simulink model "rocket_rcs"  (R2024a)
settings: Solver=FixedStepAuto  StartTime=0.0001  StopTime=140  FixedStep=0.0001  RelTol=1e-3
undefined symbols (not defined in the file or in its folder): deg, Earth, rad, s, WGS84
libraries: aerolibconvert2 x26, matrix_library x5, eePwmGenerator x5, slpidlib x5, aerolibasang x2, simulink x2, sharedtransform x1, aerolibtransform2 x1, shared6dof x1
(part 2 of 2)

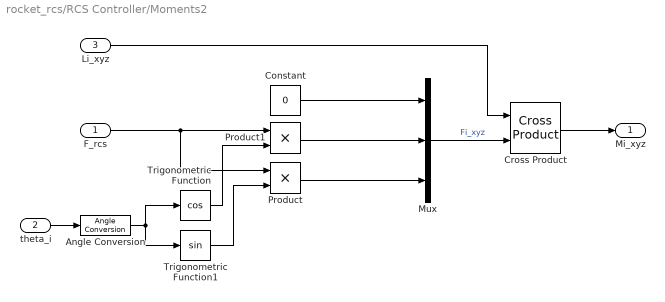
== system rocket_rcs/RCS Controller/Moments2 ==
  F_rcs : Inport
  theta_i : Inport  Port=2
  Li_xyz : Inport  Port=3
  Angle Conversion : aerolibconvert2/Angle Conversion  IU=deg  OU=rad
  Constant : Constant  Value=0
  Cross Product : matrix_library/Cross Product
  Mux : Mux  Inputs=3
  Product : Product
  Product1 : Product
  Trigonometric Function : Trigonometry  Operator=cos
  Trigonometric Function1 : Trigonometry
  Mi_xyz : Outport
  wires:
  Product1/1 -> Mux/2
  Product/1 -> Mux/3
  F_rcs/1 -> Product/1, Product1/1
  Trigonometric Function/1 -> Product1/2
  Trigonometric Function1/1 -> Product/2
  Constant/1 -> Mux/1
  Mux/1 -> Cross Product/2  "Fi_xyz"
  Li_xyz/1 -> Cross Product/1
  Cross Product/1 -> Mi_xyz/1
  theta_i/1 -> Angle Conversion/1
  Angle Conversion/1 -> Trigonometric Function1/1, Trigonometric Function/1

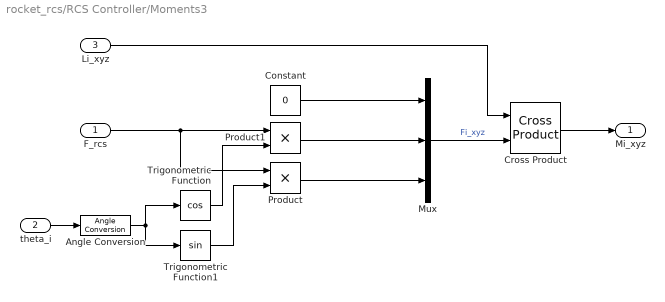
== system rocket_rcs/RCS Controller/Moments3 ==
  F_rcs : Inport
  theta_i : Inport  Port=2
  Li_xyz : Inport  Port=3
  Angle Conversion : aerolibconvert2/Angle Conversion  IU=deg  OU=rad
  Constant : Constant  Value=0
  Cross Product : matrix_library/Cross Product
  Mux : Mux  Inputs=3
  Product : Product
  Product1 : Product
  Trigonometric Function : Trigonometry  Operator=cos
  Trigonometric Function1 : Trigonometry
  Mi_xyz : Outport
  wires:
  Product1/1 -> Mux/2
  Product/1 -> Mux/3
  F_rcs/1 -> Product/1, Product1/1
  Trigonometric Function/1 -> Product1/2
  Trigonometric Function1/1 -> Product/2
  Constant/1 -> Mux/1
  Mux/1 -> Cross Product/2  "Fi_xyz"
  Li_xyz/1 -> Cross Product/1
  Cross Product/1 -> Mi_xyz/1
  theta_i/1 -> Angle Conversion/1
  Angle Conversion/1 -> Trigonometric Function1/1, Trigonometric Function/1

== system rocket_rcs/RCS Controller/PWM示例 ==
  Abs1 : Abs  SaturateOnIntegerOverflow=off
  Dead Zone2 : DeadZone  LowerValue=-0.05  UpperValue=0.05
  Divide : Product  Inputs=*/
  Dot Product : DotProduct  OutDataTypeStr=Inherit: Inherit via internal rule
  Dot Product1 : DotProduct  OutDataTypeStr=Inherit: Inherit via internal rule
  Mrcs : Constant  Value=490
  PWM Generator : eePwmGenerator/PWM Generator  CarrCount=Up  Tper=0.2  Tdelay=0  Ts=0
  Saturation : Saturate  UpperLimit=1  LowerLimit=-1
  Sign : Signum
  Sine Wave1 : Sin  Amplitude=490  Frequency=pi/2  SampleTime=0
  wires:
  Sine Wave1/1 -> Sign/1, Divide/1  "Mc"
  Sign/1 -> Dot Product/1
  Dot Product/1 -> Dot Product1/2
  Saturation/1 -> PWM Generator/1
  PWM Generator/1 -> Dot Product1/1  "PWM"
  Abs1/1 -> Dead Zone2/1
  Mrcs/1 -> Dot Product/2, Divide/2
  Divide/1 -> Abs1/1
  Dead Zone2/1 -> Saturation/1

== matlab function rocket_rcs/RCS Controller/RCS select1 ==
  data: dm_roll input; u1 output; u2 output; u3 output; u4 output; dm_pitch input; dm_raw input
% RCS 喷管选择逻辑：查表控制
function [u1,u2,u3,u4] = RCSselect(dm_roll, dm_pitch, dm_raw)

if dm_pitch < 0 && dm_raw < 0 && dm_roll < 0
    u1 = 0;
    u2 = 1;
    u3 = 1;
    u4 = 1;
elseif dm_pitch < 0 && dm_raw < 0 && dm_roll == 0
    u1 = 0;
    u2 = 0;
    u3 = 0;
    u4 = 1;
elseif dm_pitch < 0 && dm_raw < 0 && dm_roll > 0
    u1 = 0;
    u2 = 0;
    u3 = 0;
    u4 = 1;
elseif dm_pitch < 0 && dm_raw == 0 && dm_roll < 0
    u1 = 0;
    u2 = 1;
    u3 = 0;
    u4 = 0;
elseif dm_pitch < 0 && dm_raw == 0 && dm_roll == 0
    u1 = 0;
    u2 = 1;
    u3 = 0;
    u4 = 1;
elseif dm_pitch < 0 && dm_raw == 0 && dm_roll > 0
    u1 = 0;
    u2 = 0;
    u3 = 0;
    u4 = 1;
elseif dm_pitch < 0 && dm_raw > 0 && dm_roll < 0
    u1 = 0;
    u2 = 1;
    u3 = 0;
    u4 = 0;
elseif dm_pitch < 0 && dm_raw > 0 && dm_roll == 0
    u1 = 0;
    u2 = 1;
    u3 = 0;
    u4 = 0;
elseif dm_pitch < 0 && dm_raw > 0 && dm_roll > 0
    u1 = 1;
    u2 = 1;
    u3 = 0;
    u4 = 1;

elseif dm_pitch == 0 && dm_raw < 0 && dm_roll < 0
    u1 = 0;
    u2 = 0;
    u3 = 1;
    u4 = 0;
elseif dm_pitch == 0 && dm_raw < 0 && dm_roll == 0
    u1 = 0;
    u2 = 0;
    u3 = 1;
    u4 = 1;
elseif dm_pitch == 0 && dm_raw < 0 && dm_roll > 0
    u1 = 0;
    u2 = 0;
    u3 = 0;
    u4 = 1;
elseif dm_pitch == 0 && dm_raw == 0 && dm_roll < 0
    u1 = 0;
    u2 = 1;
    u3 = 1;
    u4 = 0;    
elseif dm_pitch == 0 && dm_raw == 0 && dm_roll > 0
    u1 = 1;
    u2 = 0;
    u3 = 0;
    u4 = 1;  
elseif dm_pitch == 0 && dm_raw > 0 && dm_roll < 0
    u1 = 0;
    u2 = 1;
    u3 = 0;
    u4 = 0;
elseif dm_pitch == 0 && dm_raw > 0 && dm_roll == 0
    u1 = 1;
    u2 = 1;
    u3 = 0;
    u4 = 0;    
elseif dm_pitch == 0 && dm_raw > 0 && dm_roll > 0
    u1 = 1;
    u2 = 0;
    u3 = 0;
    u4 = 0;

elseif dm_pitch > 0 && dm_raw < 0 && dm_roll < 0
    u1 = 0;
    u2 = 0;
    u3 = 1;
    u4 = 0;
elseif dm_pitch > 0 && dm_raw < 0 && dm_roll == 0
    u1 = 0;
    u2 = 0;
    u3 = 1;
    u4 = 0;
elseif dm_pitch > 0 && dm_raw < 0 && dm_roll > 0
    u1 = 1;
    u2 = 0;
    u3 = 1;
    u4 = 1;
elseif dm_pitch > 0 && dm_raw == 0 && dm_roll < 0
    u1 = 0;
    u2 = 0;
    u3 = 1;
    u4 = 0;
elseif dm_pitch > 0 && dm_raw == 0 && dm_roll == 0
    u1 = 1;
    u2 = 0;
    u3 = 1;
    u4 = 0;
elseif dm_pitch > 0 && dm_raw == 0 && dm_roll > 0
    u1 = 1;
    u2 = 0;
    u3 = 0;
    u4 = 0;
elseif dm_pitch > 0 && dm_raw > 0 && dm_roll < 0
    u1 = 1;
    u2 = 1;
    u3 = 1;
    u4 = 0;
elseif dm_pitch > 0 && dm_raw > 0 && dm_roll == 0
    u1 = 1;
    u2 = 0;
    u3 = 0;
    u4 = 0;
elseif dm_pitch > 0 && dm_raw > 0 && dm_roll > 0
    u1 = 1;
    u2 = 0;
    u3 = 0;
    u4 = 0;

else
    u1 = 0;
    u2 = 0;
    u3 = 0;
    u4 = 0;

end
end

== matlab function rocket_rcs/AeroDynamics/Air Density ==
  data: h input; Rho output
function Rho = density(h)
% rho0 = 1.225;
T0 = 288.15;    % K
p0 = 101325;   % Pa
R = 287.04;
T11 = 216.65;
p11 = 22632;
h11 = 11000;
g = 9.81;

if h <= 11000
    T=T0 - 0.0065 * h;
    p = p0 * (1-0.0065*(h/T0))^5.2561;
    Rho = p / (R * T);

elseif h>11000 && h<=20000
    T = 216.65;
    p = p11 * exp(g*(h11 - h)/(R*T11));
    Rho = p / (R * T);

else
    T=216.65+0.001*(h-20000);
    Rho=0.088035*(T/216.65)^-35.1632;
end
end

== matlab function rocket_rcs/AeroDynamics/MATLAB Function2 ==
  data: alpha input; CD output; delta_a input; delta_e input; CL output; CY output; Cl output; Cm output; delta_r input; Cn output
function [CD,CL,CY,Cl,Cm,Cn]= aeroCoeffs(alpha, delta_a, delta_e, delta_r)

% 气动系数
CL_0 = -0.404;
CL_alpha = 0.0699;
CL_delE = 0.0026;

CD_0 = -0.239;
CD_alpha = 0.035;
CD_delE = 0.0021;

CY_delR = 0.0039;

Cl_delA = 0.0023;
Cl_delR = 0.0028;
Cl_r = 0.2201;

Cm_0 = -0.0151;
% Cm_0 = 0;
Cm_alpha = 0.0117;
% Cm_delE = -0.008;
Cm_delE = 0.008;
Cm_q = 0.417;

Cn_delA = 4.997e-4;
Cn_delR = 0.0041;
Cn_p = 0.142;
% 
% % 气动力系数
CL = CL_0 + CL_alpha * alpha;
CD = CD_0 + CD_alpha * alpha + CL^2;   % 待补充
CY = 0;
% 
% % 气动力矩系数
Cl = Cl_delA * delta_a + Cl_delR * delta_r;
Cm = Cm_0 + Cm_alpha * alpha + Cm_delE * delta_e;
Cn = Cn_delA * delta_a + Cn_delR * delta_r;



end

== matlab function rocket_rcs/AeroDynamics/MATLAB Function3 ==
  data: alpha input; CD output; mach input; delta_e input; CL output; CY output; Cl output; Cm output; delta_a input; delta_r input; b input; p input; q input; r input; V input; Cn output
function [CD,CL,CY,Cl,Cm,Cn]= aeroCoeffs(alpha, mach, delta_e, delta_a, delta_r , b, p, q, r, V)

% 气动系数
CL_0 = -0.404;
CL_alpha = 0.0699;
CL_delE = 0.0026;

CD_0 = -0.239;
CD_alpha = 0.035;
CD_delE = 0.0021;

CY_delR = 0.0039;

Cl_delA = 0.0023;
Cl_delR = 0.0028;
Cl_r = 0.2201;

Cm_0 = -0.0151;
Cm_alpha = 0.0117;
Cm_delE = -0.008;
Cm_q = 0.417;

Cn_delA = 4.997e-4;
Cn_delR = 0.0041;
Cn_p = 0.142;
% 
% % 气动力系数
CL = CL_0 + CL_alpha * alpha + CL_delE * delta_e;
CD = CD_0 + CD_delE * delta_e + CD_alpha * alpha;   % 待补充
CY = CY_delR * delta_r;
% 
% % 气动力矩系数
% Cl = Cl_delA * delta_a + Cl_delR * delta_r + Cl_r * (r*b/(2*V));
% Cm = Cm_0 + Cm_alpha * alpha + Cm_delE * delta_e + Cm_q * (q*b/(2*V));
% Cn = Cn_delA * delta_a + Cn_delR * delta_r + Cn_p * (p*b/(2*V));



end
